simulink model "Hexapod_PD"  (R2026a)
settings: Solver=daessc  StopTime=ref.t(end)  FixedStep=2e-5
InitFcn:
  | startup
model workspace: external: MATLAB File Hexapod_DataFile.m (data not in the file)
undefined symbols (not defined in the file or in its folder): ref, robot, smiData, vc, X, Y, Z
libraries: sm_lib x805, nesl_utility x43
(part 7 of 15)

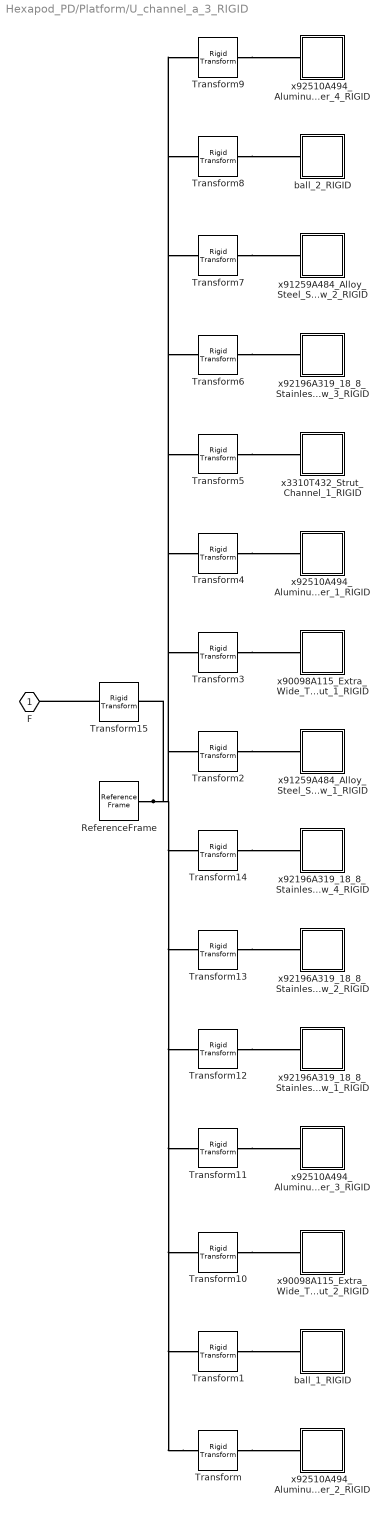
== system Hexapod_PD/Platform/U_channel_a_3_RIGID ==
  ReferenceFrame : sm_lib/Frames and Transforms/Reference Frame
  Transform : sm_lib/Frames and Transforms/Rigid Transform  RotationMethod=ArbitraryAxis  FollAlignAxisA=+X  BaseAlignAxisA=+Y  FollAlignAxisB=+Y  BaseAlignAxisB=+Z  RotationStandardAxis=+Z  RotationAngle=smiData.RigidTransform(213).angle  RotationAngleUnits=rad  RotationArbitraryAxis=smiData.RigidTransform(213).axis  RotationSequenceAxes=FollowerAxes  RotationSequence=XYX  RotationSequenceAngles=[0 0 0]  RotationSequenceAnglesUnits=deg  RotationMatrix=[1 0 0;0 1 0;0 0 1]  Quaternion=[1 0 0 0]  TranslationMethod=Cartesian  TranslationCartesianOffset=smiData.RigidTransform(213).translation  TranslationCartesianOffsetUnits=mm  TranslationStandardAxis=+Z  TranslationStandardOffset=0  TranslationStandardOffsetUnits=m  TranslationROffset=0  TranslationROffsetUnits=m  TranslationThetaOffset=0  TranslationThetaOffsetUnits=deg  TranslationZOffset=0  TranslationZOffsetUnits=m
  Transform1 : sm_lib/Frames and Transforms/Rigid Transform  RotationMethod=ArbitraryAxis  FollAlignAxisA=+X  BaseAlignAxisA=+Y  FollAlignAxisB=+Y  BaseAlignAxisB=+Z  RotationStandardAxis=+Z  RotationAngle=smiData.RigidTransform(214).angle  RotationAngleUnits=rad  RotationArbitraryAxis=smiData.RigidTransform(214).axis  RotationSequenceAxes=FollowerAxes  RotationSequence=XYX  RotationSequenceAngles=[0 0 0]  RotationSequenceAnglesUnits=deg  RotationMatrix=[1 0 0;0 1 0;0 0 1]  Quaternion=[1 0 0 0]  TranslationMethod=Cartesian  TranslationCartesianOffset=smiData.RigidTransform(214).translation  TranslationCartesianOffsetUnits=mm  TranslationStandardAxis=+Z  TranslationStandardOffset=0  TranslationStandardOffsetUnits=m  TranslationROffset=0  TranslationROffsetUnits=m  TranslationThetaOffset=0  TranslationThetaOffsetUnits=deg  TranslationZOffset=0  TranslationZOffsetUnits=m
  Transform10 : sm_lib/Frames and Transforms/Rigid Transform  RotationMethod=ArbitraryAxis  FollAlignAxisA=+X  BaseAlignAxisA=+Y  FollAlignAxisB=+Y  BaseAlignAxisB=+Z  RotationStandardAxis=+Z  RotationAngle=smiData.RigidTransform(223).angle  RotationAngleUnits=rad  RotationArbitraryAxis=smiData.RigidTransform(223).axis  RotationSequenceAxes=FollowerAxes  RotationSequence=XYX  RotationSequenceAngles=[0 0 0]  RotationSequenceAnglesUnits=deg  RotationMatrix=[1 0 0;0 1 0;0 0 1]  Quaternion=[1 0 0 0]  TranslationMethod=Cartesian  TranslationCartesianOffset=smiData.RigidTransform(223).translation  TranslationCartesianOffsetUnits=mm  TranslationStandardAxis=+Z  TranslationStandardOffset=0  TranslationStandardOffsetUnits=m  TranslationROffset=0  TranslationROffsetUnits=m  TranslationThetaOffset=0  TranslationThetaOffsetUnits=deg  TranslationZOffset=0  TranslationZOffsetUnits=m
  Transform11 : sm_lib/Frames and Transforms/Rigid Transform  RotationMethod=ArbitraryAxis  FollAlignAxisA=+X  BaseAlignAxisA=+Y  FollAlignAxisB=+Y  BaseAlignAxisB=+Z  RotationStandardAxis=+Z  RotationAngle=smiData.RigidTransform(224).angle  RotationAngleUnits=rad  RotationArbitraryAxis=smiData.RigidTransform(224).axis  RotationSequenceAxes=FollowerAxes  RotationSequence=XYX  RotationSequenceAngles=[0 0 0]  RotationSequenceAnglesUnits=deg  RotationMatrix=[1 0 0;0 1 0;0 0 1]  Quaternion=[1 0 0 0]  TranslationMethod=Cartesian  TranslationCartesianOffset=smiData.RigidTransform(224).translation  TranslationCartesianOffsetUnits=mm  TranslationStandardAxis=+Z  TranslationStandardOffset=0  TranslationStandardOffsetUnits=m  TranslationROffset=0  TranslationROffsetUnits=m  TranslationThetaOffset=0  TranslationThetaOffsetUnits=deg  TranslationZOffset=0  TranslationZOffsetUnits=m
  Transform12 : sm_lib/Frames and Transforms/Rigid Transform  RotationMethod=ArbitraryAxis  FollAlignAxisA=+X  BaseAlignAxisA=+Y  FollAlignAxisB=+Y  BaseAlignAxisB=+Z  RotationStandardAxis=+Z  RotationAngle=smiData.RigidTransform(225).angle  RotationAngleUnits=rad  RotationArbitraryAxis=smiData.RigidTransform(225).axis  RotationSequenceAxes=FollowerAxes  RotationSequence=XYX  RotationSequenceAngles=[0 0 0]  RotationSequenceAnglesUnits=deg  RotationMatrix=[1 0 0;0 1 0;0 0 1]  Quaternion=[1 0 0 0]  TranslationMethod=Cartesian  TranslationCartesianOffset=smiData.RigidTransform(225).translation  TranslationCartesianOffsetUnits=mm  TranslationStandardAxis=+Z  TranslationStandardOffset=0  TranslationStandardOffsetUnits=m  TranslationROffset=0  TranslationROffsetUnits=m  TranslationThetaOffset=0  TranslationThetaOffsetUnits=deg  TranslationZOffset=0  TranslationZOffsetUnits=m
  Transform13 : sm_lib/Frames and Transforms/Rigid Transform  RotationMethod=ArbitraryAxis  FollAlignAxisA=+X  BaseAlignAxisA=+Y  FollAlignAxisB=+Y  BaseAlignAxisB=+Z  RotationStandardAxis=+Z  RotationAngle=smiData.RigidTransform(226).angle  RotationAngleUnits=rad  RotationArbitraryAxis=smiData.RigidTransform(226).axis  RotationSequenceAxes=FollowerAxes  RotationSequence=XYX  RotationSequenceAngles=[0 0 0]  RotationSequenceAnglesUnits=deg  RotationMatrix=[1 0 0;0 1 0;0 0 1]  Quaternion=[1 0 0 0]  TranslationMethod=Cartesian  TranslationCartesianOffset=smiData.RigidTransform(226).translation  TranslationCartesianOffsetUnits=mm  TranslationStandardAxis=+Z  TranslationStandardOffset=0  TranslationStandardOffsetUnits=m  TranslationROffset=0  TranslationROffsetUnits=m  TranslationThetaOffset=0  TranslationThetaOffsetUnits=deg  TranslationZOffset=0  TranslationZOffsetUnits=m
  Transform14 : sm_lib/Frames and Transforms/Rigid Transform  RotationMethod=ArbitraryAxis  FollAlignAxisA=+X  BaseAlignAxisA=+Y  FollAlignAxisB=+Y  BaseAlignAxisB=+Z  RotationStandardAxis=+Z  RotationAngle=smiData.RigidTransform(227).angle  RotationAngleUnits=rad  RotationArbitraryAxis=smiData.RigidTransform(227).axis  RotationSequenceAxes=FollowerAxes  RotationSequence=XYX  RotationSequenceAngles=[0 0 0]  RotationSequenceAnglesUnits=deg  RotationMatrix=[1 0 0;0 1 0;0 0 1]  Quaternion=[1 0 0 0]  TranslationMethod=Cartesian  TranslationCartesianOffset=smiData.RigidTransform(227).translation  TranslationCartesianOffsetUnits=mm  TranslationStandardAxis=+Z  TranslationStandardOffset=0  TranslationStandardOffsetUnits=m  TranslationROffset=0  TranslationROffsetUnits=m  TranslationThetaOffset=0  TranslationThetaOffsetUnits=deg  TranslationZOffset=0  TranslationZOffsetUnits=m
  Transform15 : sm_lib/Frames and Transforms/Rigid Transform  RotationMethod=ArbitraryAxis  FollAlignAxisA=+X  BaseAlignAxisA=+Y  FollAlignAxisB=+Y  BaseAlignAxisB=+Z  RotationStandardAxis=+Z  RotationAngle=smiData.RigidTransform(228).angle  RotationAngleUnits=rad  RotationArbitraryAxis=smiData.RigidTransform(228).axis  RotationSequenceAxes=FollowerAxes  RotationSequence=XYX  RotationSequenceAngles=[0 0 0]  RotationSequenceAnglesUnits=deg  RotationMatrix=[1 0 0;0 1 0;0 0 1]  Quaternion=[1 0 0 0]  TranslationMethod=Cartesian  TranslationCartesianOffset=smiData.RigidTransform(228).translation  TranslationCartesianOffsetUnits=mm  TranslationStandardAxis=+Z  TranslationStandardOffset=0  TranslationStandardOffsetUnits=m  TranslationROffset=0  TranslationROffsetUnits=m  TranslationThetaOffset=0  TranslationThetaOffsetUnits=deg  TranslationZOffset=0  TranslationZOffsetUnits=m
  Transform2 : sm_lib/Frames and Transforms/Rigid Transform  RotationMethod=ArbitraryAxis  FollAlignAxisA=+X  BaseAlignAxisA=+Y  FollAlignAxisB=+Y  BaseAlignAxisB=+Z  RotationStandardAxis=+Z  RotationAngle=smiData.RigidTransform(215).angle  RotationAngleUnits=rad  RotationArbitraryAxis=smiData.RigidTransform(215).axis  RotationSequenceAxes=FollowerAxes  RotationSequence=XYX  RotationSequenceAngles=[0 0 0]  RotationSequenceAnglesUnits=deg  RotationMatrix=[1 0 0;0 1 0;0 0 1]  Quaternion=[1 0 0 0]  TranslationMethod=Cartesian  TranslationCartesianOffset=smiData.RigidTransform(215).translation  TranslationCartesianOffsetUnits=mm  TranslationStandardAxis=+Z  TranslationStandardOffset=0  TranslationStandardOffsetUnits=m  TranslationROffset=0  TranslationROffsetUnits=m  TranslationThetaOffset=0  TranslationThetaOffsetUnits=deg  TranslationZOffset=0  TranslationZOffsetUnits=m
  Transform3 : sm_lib/Frames and Transforms/Rigid Transform  RotationMethod=ArbitraryAxis  FollAlignAxisA=+X  BaseAlignAxisA=+Y  FollAlignAxisB=+Y  BaseAlignAxisB=+Z  RotationStandardAxis=+Z  RotationAngle=smiData.RigidTransform(216).angle  RotationAngleUnits=rad  RotationArbitraryAxis=smiData.RigidTransform(216).axis  RotationSequenceAxes=FollowerAxes  RotationSequence=XYX  RotationSequenceAngles=[0 0 0]  RotationSequenceAnglesUnits=deg  RotationMatrix=[1 0 0;0 1 0;0 0 1]  Quaternion=[1 0 0 0]  TranslationMethod=Cartesian  TranslationCartesianOffset=smiData.RigidTransform(216).translation  TranslationCartesianOffsetUnits=mm  TranslationStandardAxis=+Z  TranslationStandardOffset=0  TranslationStandardOffsetUnits=m  TranslationROffset=0  TranslationROffsetUnits=m  TranslationThetaOffset=0  TranslationThetaOffsetUnits=deg  TranslationZOffset=0  TranslationZOffsetUnits=m
  Transform4 : sm_lib/Frames and Transforms/Rigid Transform  RotationMethod=ArbitraryAxis  FollAlignAxisA=+X  BaseAlignAxisA=+Y  FollAlignAxisB=+Y  BaseAlignAxisB=+Z  RotationStandardAxis=+Z  RotationAngle=smiData.RigidTransform(217).angle  RotationAngleUnits=rad  RotationArbitraryAxis=smiData.RigidTransform(217).axis  RotationSequenceAxes=FollowerAxes  RotationSequence=XYX  RotationSequenceAngles=[0 0 0]  RotationSequenceAnglesUnits=deg  RotationMatrix=[1 0 0;0 1 0;0 0 1]  Quaternion=[1 0 0 0]  TranslationMethod=Cartesian  TranslationCartesianOffset=smiData.RigidTransform(217).translation  TranslationCartesianOffsetUnits=mm  TranslationStandardAxis=+Z  TranslationStandardOffset=0  TranslationStandardOffsetUnits=m  TranslationROffset=0  TranslationROffsetUnits=m  TranslationThetaOffset=0  TranslationThetaOffsetUnits=deg  TranslationZOffset=0  TranslationZOffsetUnits=m
  Transform5 : sm_lib/Frames and Transforms/Rigid Transform  RotationMethod=ArbitraryAxis  FollAlignAxisA=+X  BaseAlignAxisA=+Y  FollAlignAxisB=+Y  BaseAlignAxisB=+Z  RotationStandardAxis=+Z  RotationAngle=smiData.RigidTransform(218).angle  RotationAngleUnits=rad  RotationArbitraryAxis=smiData.RigidTransform(218).axis  RotationSequenceAxes=FollowerAxes  RotationSequence=XYX  RotationSequenceAngles=[0 0 0]  RotationSequenceAnglesUnits=deg  RotationMatrix=[1 0 0;0 1 0;0 0 1]  Quaternion=[1 0 0 0]  TranslationMethod=Cartesian  TranslationCartesianOffset=smiData.RigidTransform(218).translation  TranslationCartesianOffsetUnits=mm  TranslationStandardAxis=+Z  TranslationStandardOffset=0  TranslationStandardOffsetUnits=m  TranslationROffset=0  TranslationROffsetUnits=m  TranslationThetaOffset=0  TranslationThetaOffsetUnits=deg  TranslationZOffset=0  TranslationZOffsetUnits=m
  Transform6 : sm_lib/Frames and Transforms/Rigid Transform  RotationMethod=ArbitraryAxis  FollAlignAxisA=+X  BaseAlignAxisA=+Y  FollAlignAxisB=+Y  BaseAlignAxisB=+Z  RotationStandardAxis=+Z  RotationAngle=smiData.RigidTransform(219).angle  RotationAngleUnits=rad  RotationArbitraryAxis=smiData.RigidTransform(219).axis  RotationSequenceAxes=FollowerAxes  RotationSequence=XYX  RotationSequenceAngles=[0 0 0]  RotationSequenceAnglesUnits=deg  RotationMatrix=[1 0 0;0 1 0;0 0 1]  Quaternion=[1 0 0 0]  TranslationMethod=Cartesian  TranslationCartesianOffset=smiData.RigidTransform(219).translation  TranslationCartesianOffsetUnits=mm  TranslationStandardAxis=+Z  TranslationStandardOffset=0  TranslationStandardOffsetUnits=m  TranslationROffset=0  TranslationROffsetUnits=m  TranslationThetaOffset=0  TranslationThetaOffsetUnits=deg  TranslationZOffset=0  TranslationZOffsetUnits=m
  Transform7 : sm_lib/Frames and Transforms/Rigid Transform  RotationMethod=ArbitraryAxis  FollAlignAxisA=+X  BaseAlignAxisA=+Y  FollAlignAxisB=+Y  BaseAlignAxisB=+Z  RotationStandardAxis=+Z  RotationAngle=smiData.RigidTransform(220).angle  RotationAngleUnits=rad  RotationArbitraryAxis=smiData.RigidTransform(220).axis  RotationSequenceAxes=FollowerAxes  RotationSequence=XYX  RotationSequenceAngles=[0 0 0]  RotationSequenceAnglesUnits=deg  RotationMatrix=[1 0 0;0 1 0;0 0 1]  Quaternion=[1 0 0 0]  TranslationMethod=Cartesian  TranslationCartesianOffset=smiData.RigidTransform(220).translation  TranslationCartesianOffsetUnits=mm  TranslationStandardAxis=+Z  TranslationStandardOffset=0  TranslationStandardOffsetUnits=m  TranslationROffset=0  TranslationROffsetUnits=m  TranslationThetaOffset=0  TranslationThetaOffsetUnits=deg  TranslationZOffset=0  TranslationZOffsetUnits=m
  Transform8 : sm_lib/Frames and Transforms/Rigid Transform  RotationMethod=ArbitraryAxis  FollAlignAxisA=+X  BaseAlignAxisA=+Y  FollAlignAxisB=+Y  BaseAlignAxisB=+Z  RotationStandardAxis=+Z  RotationAngle=smiData.RigidTransform(221).angle  RotationAngleUnits=rad  RotationArbitraryAxis=smiData.RigidTransform(221).axis  RotationSequenceAxes=FollowerAxes  RotationSequence=XYX  RotationSequenceAngles=[0 0 0]  RotationSequenceAnglesUnits=deg  RotationMatrix=[1 0 0;0 1 0;0 0 1]  Quaternion=[1 0 0 0]  TranslationMethod=Cartesian  TranslationCartesianOffset=smiData.RigidTransform(221).translation  TranslationCartesianOffsetUnits=mm  TranslationStandardAxis=+Z  TranslationStandardOffset=0  TranslationStandardOffsetUnits=m  TranslationROffset=0  TranslationROffsetUnits=m  TranslationThetaOffset=0  TranslationThetaOffsetUnits=deg  TranslationZOffset=0  TranslationZOffsetUnits=m
  Transform9 : sm_lib/Frames and Transforms/Rigid Transform  RotationMethod=ArbitraryAxis  FollAlignAxisA=+X  BaseAlignAxisA=+Y  FollAlignAxisB=+Y  BaseAlignAxisB=+Z  RotationStandardAxis=+Z  RotationAngle=smiData.RigidTransform(222).angle  RotationAngleUnits=rad  RotationArbitraryAxis=smiData.RigidTransform(222).axis  RotationSequenceAxes=FollowerAxes  RotationSequence=XYX  RotationSequenceAngles=[0 0 0]  RotationSequenceAnglesUnits=deg  RotationMatrix=[1 0 0;0 1 0;0 0 1]  Quaternion=[1 0 0 0]  TranslationMethod=Cartesian  TranslationCartesianOffset=smiData.RigidTransform(222).translation  TranslationCartesianOffsetUnits=mm  TranslationStandardAxis=+Z  TranslationStandardOffset=0  TranslationStandardOffsetUnits=m  TranslationROffset=0  TranslationROffsetUnits=m  TranslationThetaOffset=0  TranslationThetaOffsetUnits=deg  TranslationZOffset=0  TranslationZOffsetUnits=m
  ball_1_RIGID : Subsystem
  ball_2_RIGID : Subsystem
  x3310T432_Strut_Channel_1_RIGID : Subsystem
  x90098A115_Extra_Wide_Thin_Nylon_Insert_Locknut_1_RIGID : Subsystem
  x90098A115_Extra_Wide_Thin_Nylon_Insert_Locknut_2_RIGID : Subsystem
  x91259A484_Alloy_Steel_Shoulder_Screw_1_RIGID : Subsystem
  x91259A484_Alloy_Steel_Shoulder_Screw_2_RIGID : Subsystem
  x92196A319_18_8_Stainless_Steel_Socket_Head_Screw_1_RIGID : Subsystem
  x92196A319_18_8_Stainless_Steel_Socket_Head_Screw_2_RIGID : Subsystem
  x92196A319_18_8_Stainless_Steel_Socket_Head_Screw_3_RIGID : Subsystem
  x92196A319_18_8_Stainless_Steel_Socket_Head_Screw_4_RIGID : Subsystem
  x92510A494_Aluminum_Unthreaded_Spacer_1_RIGID : Subsystem
  x92510A494_Aluminum_Unthreaded_Spacer_2_RIGID : Subsystem
  x92510A494_Aluminum_Unthreaded_Spacer_3_RIGID : Subsystem
  x92510A494_Aluminum_Unthreaded_Spacer_4_RIGID : Subsystem
  F : PMIOPort  Side=Right
  connections:
  Transform/RConn1 -- x92510A494_Aluminum_Unthreaded_Spacer_2_RIGID/LConn1
  Transform1/RConn1 -- ball_1_RIGID/LConn1
  Transform10/RConn1 -- x90098A115_Extra_Wide_Thin_Nylon_Insert_Locknut_2_RIGID/LConn1
  Transform11/RConn1 -- x92510A494_Aluminum_Unthreaded_Spacer_3_RIGID/LConn1
  Transform12/RConn1 -- x92196A319_18_8_Stainless_Steel_Socket_Head_Screw_1_RIGID/LConn1
  Transform13/RConn1 -- x92196A319_18_8_Stainless_Steel_Socket_Head_Screw_2_RIGID/LConn1
  Transform14/RConn1 -- x92196A319_18_8_Stainless_Steel_Socket_Head_Screw_4_RIGID/LConn1
  Transform/LConn1 -- ReferenceFrame/RConn1 -- Transform1/LConn1 -- Transform10/LConn1 -- Transform11/LConn1 -- Transform12/LConn1 -- Transform13/LConn1 -- Transform14/LConn1 -- Transform15/RConn1 -- Transform2/LConn1 -- Transform3/LConn1 -- Transform4/LConn1 -- Transform5/LConn1 -- Transform6/LConn1 -- Transform7/LConn1 -- Transform8/LConn1 -- Transform9/LConn1
  Transform15/LConn1 -- F/RConn1
  Transform2/RConn1 -- x91259A484_Alloy_Steel_Shoulder_Screw_1_RIGID/LConn1
  Transform3/RConn1 -- x90098A115_Extra_Wide_Thin_Nylon_Insert_Locknut_1_RIGID/LConn1
  Transform4/RConn1 -- x92510A494_Aluminum_Unthreaded_Spacer_1_RIGID/LConn1
  Transform5/RConn1 -- x3310T432_Strut_Channel_1_RIGID/LConn1
  Transform6/RConn1 -- x92196A319_18_8_Stainless_Steel_Socket_Head_Screw_3_RIGID/LConn1
  Transform7/RConn1 -- x91259A484_Alloy_Steel_Shoulder_Screw_2_RIGID/LConn1
  Transform8/RConn1 -- ball_2_RIGID/LConn1
  Transform9/RConn1 -- x92510A494_Aluminum_Unthreaded_Spacer_4_RIGID/LConn1

== system Hexapod_PD/Platform pose logger/g ==
  Ina : Inport
  Demux : Demux  Outputs=3
  Mux1 : Mux  Inputs=3
  g : Bias  Bias=robot.g  SaturateOnIntegerOverflow=off
  Outa : Outport
  wires:
  Demux/1 -> Mux1/1
  Demux/3 -> g/1
  Mux1/1 -> Outa/1
  g/1 -> Mux1/3
  Demux/2 -> Mux1/2
  Ina/1 -> Demux/1

== system Hexapod_PD/Revolute Joints/PD controller1 ==
  clock : Inport
  Add : Sum
  Constant : Constant  Value=deg2rad(smiData.RevoluteJoint(1).Rz.Pos)
  D gain : Gain  Gain=vc.Kd
  Differentiator : TransferFcn  Numerator=[vc.wf 0]  Denominator=[1 vc.wf]
  FF gin : Gain  Gain=vc.Kv
  Gain : Gain  Gain=-1
  Integrator : Integrator
  P gain : Gain  Gain=vc.Kp
  Sum : Sum  Inputs=|++-
  Sum1 : Sum  Inputs=|+-
  Velocity Plant : TransferFcn  Numerator=[robot.drive.a]  Denominator=[1 robot.drive.b]
  du : Lookup_n-D  NumberOfTableDimensions=1  BreakpointsForDimension1=ref.t  Table=ref.qd(:,1)  InterpMethod=Cubic spline  InternalRulePriority=Speed  RndMeth=Simplest
  u : Lookup_n-D  NumberOfTableDimensions=1  BreakpointsForDimension1=ref.t  Table=ref.q(:,1)  InterpMethod=Cubic spline  InternalRulePriority=Speed  RndMeth=Simplest
  y : Outport
  wires:
  P gain/1 -> Sum/2
  Sum/1 -> Velocity Plant/1
  Sum1/1 -> P gain/1
  Velocity Plant/1 -> Integrator/1
  D gain/1 -> Sum/3
  Differentiator/1 -> D gain/1
  du/1 -> FF gin/1  "omega ref"
  FF gin/1 -> Sum/1
  clock/1 -> u/1, du/1
  u/1 -> Sum1/1  "theta ref"
  Integrator/1 -> Gain/1, Sum1/2, Differentiator/1
  Add/1 -> y/1
  Gain/1 -> Add/2
  Constant/1 -> Add/1

== system Hexapod_PD/Revolute Joints/PD controller2 ==
  clock : Inport
  Add : Sum
  Constant : Constant  Value=deg2rad(smiData.RevoluteJoint(2).Rz.Pos)
  D gain : Gain  Gain=vc.Kd
  Differentiator : TransferFcn  Numerator=[vc.wf 0]  Denominator=[1 vc.wf]
  FF gin : Gain  Gain=vc.Kv
  Gain : Gain
  Integrator : Integrator
  P gain : Gain  Gain=vc.Kp
  Sum : Sum  Inputs=|++-
  Sum1 : Sum  Inputs=|+-
  Velocity Plant : TransferFcn  Numerator=[robot.drive.a]  Denominator=[1 robot.drive.b]
  du : Lookup_n-D  NumberOfTableDimensions=1  BreakpointsForDimension1=ref.t  Table=ref.qd(:,2)  InterpMethod=Cubic spline  InternalRulePriority=Speed  RndMeth=Simplest
  u : Lookup_n-D  NumberOfTableDimensions=1  BreakpointsForDimension1=ref.t  Table=ref.q(:,2)  InterpMethod=Cubic spline  InternalRulePriority=Speed  RndMeth=Simplest
  y : Outport
  wires:
  P gain/1 -> Sum/2
  Sum/1 -> Velocity Plant/1
  Sum1/1 -> P gain/1
  Velocity Plant/1 -> Integrator/1
  D gain/1 -> Sum/3
  Differentiator/1 -> D gain/1
  du/1 -> FF gin/1  "v ref"
  FF gin/1 -> Sum/1
  clock/1 -> u/1, du/1
  u/1 -> Sum1/1
  Integrator/1 -> Gain/1, Sum1/2, Differentiator/1
  Gain/1 -> Add/1
  Constant/1 -> Add/2
  Add/1 -> y/1

== system Hexapod_PD/Revolute Joints/PD controller3 ==
  clock : Inport
  Add : Sum
  Constant : Constant  Value=deg2rad(smiData.RevoluteJoint(5).Rz.Pos)
  D gain : Gain  Gain=vc.Kd
  Differentiator : TransferFcn  Numerator=[vc.wf 0]  Denominator=[1 vc.wf]
  FF gin : Gain  Gain=vc.Kv
  Gain : Gain  Gain=-1
  Integrator : Integrator
  P gain : Gain  Gain=vc.Kp
  Sum : Sum  Inputs=|++-
  Sum1 : Sum  Inputs=|+-
  Velocity Plant : TransferFcn  Numerator=[robot.drive.a]  Denominator=[1 robot.drive.b]
  du : Lookup_n-D  NumberOfTableDimensions=1  BreakpointsForDimension1=ref.t  Table=ref.qd(:,3)  InterpMethod=Cubic spline  InternalRulePriority=Speed  RndMeth=Simplest
  u : Lookup_n-D  NumberOfTableDimensions=1  BreakpointsForDimension1=ref.t  Table=ref.q(:,3)  InterpMethod=Cubic spline  InternalRulePriority=Speed  RndMeth=Simplest
  y : Outport
  wires:
  P gain/1 -> Sum/2
  Sum/1 -> Velocity Plant/1
  Sum1/1 -> P gain/1
  Velocity Plant/1 -> Integrator/1
  D gain/1 -> Sum/3
  Differentiator/1 -> D gain/1
  du/1 -> FF gin/1  "v ref"
  FF gin/1 -> Sum/1
  clock/1 -> u/1, du/1
  u/1 -> Sum1/1
  Integrator/1 -> Gain/1, Sum1/2, Differentiator/1
  Gain/1 -> Add/1
  Constant/1 -> Add/2
  Add/1 -> y/1

== system Hexapod_PD/Revolute Joints/PD controller4 ==
  clock : Inport
  Add : Sum
  Constant : Constant  Value=deg2rad(smiData.RevoluteJoint(6).Rz.Pos)
  D gain : Gain  Gain=vc.Kd
  Differentiator : TransferFcn  Numerator=[vc.wf 0]  Denominator=[1 vc.wf]
  FF gin : Gain  Gain=vc.Kv
  Gain : Gain
  Integrator : Integrator
  P gain : Gain  Gain=vc.Kp
  Sum : Sum  Inputs=|++-
  Sum1 : Sum  Inputs=|+-
  Velocity Plant : TransferFcn  Numerator=[robot.drive.a]  Denominator=[1 robot.drive.b]
  du : Lookup_n-D  NumberOfTableDimensions=1  BreakpointsForDimension1=ref.t  Table=ref.qd(:,4)  InterpMethod=Cubic spline  InternalRulePriority=Speed  RndMeth=Simplest
  u : Lookup_n-D  NumberOfTableDimensions=1  BreakpointsForDimension1=ref.t  Table=ref.q(:,4)  InterpMethod=Cubic spline  InternalRulePriority=Speed  RndMeth=Simplest
  y : Outport
  wires:
  P gain/1 -> Sum/2
  Sum/1 -> Velocity Plant/1
  Sum1/1 -> P gain/1
  Velocity Plant/1 -> Integrator/1
  D gain/1 -> Sum/3
  Differentiator/1 -> D gain/1
  du/1 -> FF gin/1  "v ref"
  FF gin/1 -> Sum/1
  clock/1 -> u/1, du/1
  u/1 -> Sum1/1
  Integrator/1 -> Gain/1, Sum1/2, Differentiator/1
  Gain/1 -> Add/1
  Constant/1 -> Add/2
  Add/1 -> y/1

== system Hexapod_PD/Revolute Joints/PD controller5 ==
  clock : Inport
  Add : Sum
  Constant : Constant  Value=deg2rad(smiData.RevoluteJoint(3).Rz.Pos)
  D gain : Gain  Gain=vc.Kd
  Differentiator : TransferFcn  Numerator=[vc.wf 0]  Denominator=[1 vc.wf]
  FF gin : Gain  Gain=vc.Kv
  Gain : Gain  Gain=-1
  Integrator : Integrator
  P gain : Gain  Gain=vc.Kp
  Sum : Sum  Inputs=|++-
  Sum1 : Sum  Inputs=|+-
  Velocity Plant : TransferFcn  Numerator=[robot.drive.a]  Denominator=[1 robot.drive.b]
  du : Lookup_n-D  NumberOfTableDimensions=1  BreakpointsForDimension1=ref.t  Table=ref.qd(:,5)  InterpMethod=Cubic spline  InternalRulePriority=Speed  RndMeth=Simplest
  u : Lookup_n-D  NumberOfTableDimensions=1  BreakpointsForDimension1=ref.t  Table=ref.q(:,5)  InterpMethod=Cubic spline  InternalRulePriority=Speed  RndMeth=Simplest
  y : Outport
  wires:
  P gain/1 -> Sum/2
  Sum/1 -> Velocity Plant/1
  Sum1/1 -> P gain/1
  Velocity Plant/1 -> Integrator/1
  D gain/1 -> Sum/3
  Differentiator/1 -> D gain/1
  du/1 -> FF gin/1  "v ref"
  FF gin/1 -> Sum/1
  clock/1 -> u/1, du/1
  u/1 -> Sum1/1
  Integrator/1 -> Gain/1, Sum1/2, Differentiator/1
  Gain/1 -> Add/1
  Constant/1 -> Add/2
  Add/1 -> y/1

== system Hexapod_PD/Revolute Joints/PD controller6 ==
  clock : Inport
  Add : Sum
  Constant : Constant  Value=deg2rad(smiData.RevoluteJoint(4).Rz.Pos)
  D gain : Gain  Gain=vc.Kd
  Differentiator : TransferFcn  Numerator=[vc.wf 0]  Denominator=[1 vc.wf]
  FF gin : Gain  Gain=vc.Kv
  Gain : Gain
  Integrator : Integrator
  P gain : Gain  Gain=vc.Kp
  Sum : Sum  Inputs=|++-
  Sum1 : Sum  Inputs=|+-
  Velocity Plant : TransferFcn  Numerator=[robot.drive.a]  Denominator=[1 robot.drive.b]
  du : Lookup_n-D  NumberOfTableDimensions=1  BreakpointsForDimension1=ref.t  Table=ref.qd(:,6)  InterpMethod=Cubic spline  InternalRulePriority=Speed  RndMeth=Simplest
  u : Lookup_n-D  NumberOfTableDimensions=1  BreakpointsForDimension1=ref.t  Table=ref.q(:,6)  InterpMethod=Cubic spline  InternalRulePriority=Speed  RndMeth=Simplest
  y : Outport
  wires:
  P gain/1 -> Sum/2
  Sum/1 -> Velocity Plant/1
  Sum1/1 -> P gain/1
  Velocity Plant/1 -> Integrator/1
  D gain/1 -> Sum/3
  Differentiator/1 -> D gain/1
  du/1 -> FF gin/1  "v ref"
  FF gin/1 -> Sum/1
  clock/1 -> u/1, du/1
  u/1 -> Sum1/1
  Integrator/1 -> Gain/1, Sum1/2, Differentiator/1
  Gain/1 -> Add/1
  Constant/1 -> Add/2
  Add/1 -> y/1

== system Hexapod_PD/Revolute Joints/Subsystem ==
  Gain2 : Gain  Gain=-1
  MotorFrametoBodyFrame3 : Subsystem
  Mux2 : Mux
  PS-Simulink Converter{8..11} (4 alike) : nesl_utility/PS-Simulink Converter  PhysicalDomain=network_engine_domain  SubClassName=ps_output  LeftPortType=input  RightPortType=output  PseudoPeriodic=off  Frequencies=[]  VectorFormat=inherit  Unit=inherit  AffineConversion=off
  q : PMIOPort  Side=Left
  w : PMIOPort  Port=2  Side=Left
  b : PMIOPort  Port=3  Side=Left
  t : PMIOPort  Port=4  Side=Left
  3 : Outport
  wires:
  PS-Simulink Converter8/1 -> MotorFrametoBodyFrame3/1(M)
  PS-Simulink Converter9/1 -> Mux2/2
  PS-Simulink Converter10/1 -> Mux2/3
  MotorFrametoBodyFrame3/1(B) -> Mux2/1
  Mux2/1 -> Gain2/1
  PS-Simulink Converter11/1 -> Mux2/4
  Gain2/1 -> 3/1
  connections:
  t/RConn1 -- PS-Simulink Converter11/LConn1
  b/RConn1 -- PS-Simulink Converter10/LConn1
  q/RConn1 -- PS-Simulink Converter8/LConn1
  w/RConn1 -- PS-Simulink Converter9/LConn1

== system Hexapod_PD/Revolute Joints/Subsystem10 ==
  Gain3 : Gain  Gain=-1
  MotorFrametoBodyFrame5 : Subsystem
  Mux4 : Mux
  PS-Simulink Converter{16..19} (4 alike) : nesl_utility/PS-Simulink Converter  PhysicalDomain=network_engine_domain  SubClassName=ps_output  LeftPortType=input  RightPortType=output  PseudoPeriodic=off  Frequencies=[]  VectorFormat=inherit  Unit=inherit  AffineConversion=off
  q : PMIOPort  Side=Left
  w : PMIOPort  Port=2  Side=Left
  b : PMIOPort  Port=3  Side=Left
  t : PMIOPort  Port=4  Side=Left
  5 : Outport
  wires:
  PS-Simulink Converter17/1 -> Mux4/4
  PS-Simulink Converter16/1 -> Mux4/3
  Mux4/1 -> Gain3/1
  PS-Simulink Converter18/1 -> MotorFrametoBodyFrame5/1(M)
  PS-Simulink Converter19/1 -> Mux4/2
  MotorFrametoBodyFrame5/1(B) -> Mux4/1
  Gain3/1 -> 5/1
  connections:
  w/RConn1 -- PS-Simulink Converter19/LConn1
  t/RConn1 -- PS-Simulink Converter17/LConn1
  b/RConn1 -- PS-Simulink Converter16/LConn1
  q/RConn1 -- PS-Simulink Converter18/LConn1

== system Hexapod_PD/Revolute Joints/Subsystem11 ==
  MotorFrametoBodyFrame6 : Subsystem
  Mux5 : Mux
  PS-Simulink Converter{20..23} (4 alike) : nesl_utility/PS-Simulink Converter  PhysicalDomain=network_engine_domain  SubClassName=ps_output  LeftPortType=input  RightPortType=output  PseudoPeriodic=off  Frequencies=[]  VectorFormat=inherit  Unit=inherit  AffineConversion=off
  q : PMIOPort  Side=Left
  w : PMIOPort  Port=2  Side=Left
  b : PMIOPort  Port=3  Side=Left
  t : PMIOPort  Port=4  Side=Left
  6 : Outport
  wires:
  PS-Simulink Converter20/1 -> Mux5/3
  PS-Simulink Converter23/1 -> Mux5/2
  PS-Simulink Converter21/1 -> Mux5/4
  PS-Simulink Converter22/1 -> MotorFrametoBodyFrame6/1(M)
  MotorFrametoBodyFrame6/1(B) -> Mux5/1
  Mux5/1 -> 6/1
  connections:
  w/RConn1 -- PS-Simulink Converter23/LConn1
  t/RConn1 -- PS-Simulink Converter21/LConn1
  q/RConn1 -- PS-Simulink Converter22/LConn1
  b/RConn1 -- PS-Simulink Converter20/LConn1

== system Hexapod_PD/Revolute Joints/Subsystem7 ==
  Gain1 : Gain  Gain=-1
  MotorFrametoBodyFrame1 : Subsystem
  Mux : Mux
  PS-Simulink Converter{,1..3} (4 alike) : nesl_utility/PS-Simulink Converter  PhysicalDomain=network_engine_domain  SubClassName=ps_output  LeftPortType=input  RightPortType=output  PseudoPeriodic=off  Frequencies=[]  VectorFormat=inherit  Unit=inherit  AffineConversion=off
  q : PMIOPort  Side=Left
  w : PMIOPort  Port=2  Side=Left
  b : PMIOPort  Port=3  Side=Left
  t : PMIOPort  Port=4  Side=Left
  1 : Outport
  wires:
  Mux/1 -> Gain1/1
  PS-Simulink Converter/1 -> MotorFrametoBodyFrame1/1(M)
  PS-Simulink Converter3/1 -> Mux/4
  MotorFrametoBodyFrame1/1(B) -> Mux/1
  PS-Simulink Converter2/1 -> Mux/3
  Gain1/1 -> 1/1
  PS-Simulink Converter1/1 -> Mux/2
  connections:
  w/RConn1 -- PS-Simulink Converter1/LConn1
  q/RConn1 -- PS-Simulink Converter/LConn1
  t/RConn1 -- PS-Simulink Converter3/LConn1
  b/RConn1 -- PS-Simulink Converter2/LConn1

== system Hexapod_PD/Revolute Joints/Subsystem8 ==
  MotorFrametoBodyFrame2 : Subsystem
  Mux1 : Mux
  PS-Simulink Converter{4..7} (4 alike) : nesl_utility/PS-Simulink Converter  PhysicalDomain=network_engine_domain  SubClassName=ps_output  LeftPortType=input  RightPortType=output  PseudoPeriodic=off  Frequencies=[]  VectorFormat=inherit  Unit=inherit  AffineConversion=off
  q : PMIOPort  Side=Left
  w : PMIOPort  Port=2  Side=Left
  b : PMIOPort  Port=3  Side=Left
  t : PMIOPort  Port=4  Side=Left
  2 : Outport
  wires:
  MotorFrametoBodyFrame2/1(B) -> Mux1/1
  PS-Simulink Converter4/1 -> MotorFrametoBodyFrame2/1(M)
  PS-Simulink Converter6/1 -> Mux1/3
  PS-Simulink Converter5/1 -> Mux1/2
  PS-Simulink Converter7/1 -> Mux1/4
  Mux1/1 -> 2/1
  connections:
  q/RConn1 -- PS-Simulink Converter4/LConn1
  w/RConn1 -- PS-Simulink Converter5/LConn1
  b/RConn1 -- PS-Simulink Converter6/LConn1
  t/RConn1 -- PS-Simulink Converter7/LConn1

== system Hexapod_PD/Revolute Joints/Subsystem9 ==
  MotorFrametoBodyFrame4 : Subsystem
  Mux3 : Mux
  PS-Simulink Converter{12..15} (4 alike) : nesl_utility/PS-Simulink Converter  PhysicalDomain=network_engine_domain  SubClassName=ps_output  LeftPortType=input  RightPortType=output  PseudoPeriodic=off  Frequencies=[]  VectorFormat=inherit  Unit=inherit  AffineConversion=off
  q : PMIOPort  Side=Left
  w : PMIOPort  Port=2  Side=Left
  b : PMIOPort  Port=3  Side=Left
  t : PMIOPort  Port=4  Side=Left
  4 : Outport
  wires:
  PS-Simulink Converter12/1 -> Mux3/3
  PS-Simulink Converter15/1 -> Mux3/2
  PS-Simulink Converter13/1 -> Mux3/4
  PS-Simulink Converter14/1 -> MotorFrametoBodyFrame4/1(M)
  MotorFrametoBodyFrame4/1(B) -> Mux3/1
  Mux3/1 -> 4/1
  connections:
  w/RConn1 -- PS-Simulink Converter15/LConn1
  t/RConn1 -- PS-Simulink Converter13/LConn1
  q/RConn1 -- PS-Simulink Converter14/LConn1
  b/RConn1 -- PS-Simulink Converter12/LConn1

== system Hexapod_PD/Spherical Joints/HeimJoint_No_Ball_1_RIGID1 ==
  ReferenceFrame : sm_lib/Frames and Transforms/Reference Frame
  Solid : sm_lib/Body Elements/File Solid  ExtGeomFileName=6960T431_Super-Swivel Ball Joint Rod End No Ball_6960T431_sldprt.STEP  UnitType=FromFile  ExtGeomFileUnits=m  StepReaderType=HEX  ExportConvexHullGeometry=off  InertiaType=Custom  BasedOnType=DensityFromFile  Density=1000  DensityUnits=kg/m^3  Mass=smiData.Solid(20).mass  MassUnits=kg  CenterOfMass=smiData.Solid(20).CoM  CenterOfMassUnits=in  MomentsOfInertia=smiData.Solid(20).MoI  MomentsOfInertiaUnits=kg*in^2  ProductsOfInertia=smiData.Solid(20).PoI  ProductsOfInertiaUnits=kg*in^2  GraphicType=FromGeometry  MarkerShape=Sphere  MarkerSize=10  GraphicVisPropType=SimpleVisualProperties  GraphicDiffuseColor=smiData.Solid(20).color  GraphicOpacity=smiData.Solid(20).opacity  GraphicSpecularColor=[0.5 0.5 0.5 1.0]  GraphicAmbientColor=[0.15 0.15 0.15 1.0]  GraphicEmissiveColor=[0.0 0.0 0.0 1.0]  GraphicShininess=75  DoExposeReferenceFrame=on  SerializedFrames=|
      | <Frames>
      | 
      |   <Frame>
      |     <Id>Frame1</Id>
      |     <Value>
      |       <Name>B</Name>
      |       <Origin>
      |         <Source>GeometricFeature</Source>
      |         <FeatureName>circular curve 99</FeatureName>
      |       </Origin>
      |       <PrimaryAxis>
      |         <DefinedDirection>+Z</DefinedDirection>
      |         <Source>ReferenceFrame</Source>
      |         <SourceDirection>+Z</SourceDirection>
      |         <FeatureName></FeatureName>
      |       </PrimaryAxis>
      |       <SecondaryAxis>
      |         <DefinedDirection>-X</DefinedDirection>
      |         <Source>GeometricFeature</Source>
      |         <SourceDirection>+X</SourceDirection>
      |         <FeatureName>segment 73</FeatureName>
      |       </SecondaryAxis>
      |     </Value>
      |   </Frame>
      | 
      | </Frames>
  Solid1 : sm_lib/Body Elements/File Solid  ExtGeomFileName=6960T432_Super-Swivel Ball Joint Rod End No Ball_6960T432_sldprt.STEP  UnitType=FromFile  ExtGeomFileUnits=m  StepReaderType=HEX  ExportConvexHullGeometry=off  InertiaType=Custom  BasedOnType=DensityFromFile  Density=1000  DensityUnits=kg/m^3  Mass=smiData.Solid(21).mass  MassUnits=kg  CenterOfMass=smiData.Solid(21).CoM  CenterOfMassUnits=in  MomentsOfInertia=smiData.Solid(21).MoI  MomentsOfInertiaUnits=kg*in^2  ProductsOfInertia=smiData.Solid(21).PoI  ProductsOfInertiaUnits=kg*in^2  GraphicType=FromGeometry  MarkerShape=Sphere  MarkerSize=10  GraphicVisPropType=SimpleVisualProperties  GraphicDiffuseColor=smiData.Solid(21).color  GraphicOpacity=smiData.Solid(21).opacity  GraphicSpecularColor=[0.5 0.5 0.5 1.0]  GraphicAmbientColor=[0.15 0.15 0.15 1.0]  GraphicEmissiveColor=[0.0 0.0 0.0 1.0]  GraphicShininess=75  DoExposeReferenceFrame=on  SerializedFrames=|
      | <Frames>
      | 
      |   <Frame>
      |     <Id>Frame1</Id>
      |     <Value>
      |       <Name>T</Name>
      |       <Origin>
      |         <Source>GeometricFeature</Source>
      |         <FeatureName>spherical surface 2</FeatureName>
      |       </Origin>
      |       <PrimaryAxis>
      |         <DefinedDirection>+Z</DefinedDirection>
      |         <Source>ReferenceFrame</Source>
      |         <SourceDirection>+Z</SourceDirection>
      |         <FeatureName></FeatureName>
      |       </PrimaryAxis>
      |       <SecondaryAxis>
      |         <DefinedDirection>+X</DefinedDirection>
      |         <Source>GeometricFeature</Source>
      |         <SourceDirection>+X</SourceDirection>
      |         <FeatureName>segment 75</FeatureName>
      |       </SecondaryAxis>
      |     </Value>
      |   </Frame>
      | 
      | </Frames>
  Solid2 : sm_lib/Body Elements/File Solid  ExtGeomFileName=8422N111_18-8 Stainless Steel Turnbuckle-Style Connecting Rod_8422N111_sldprt.STEP  UnitType=FromFile  ExtGeomFileUnits=m  StepReaderType=HEX  ExportConvexHullGeometry=off  InertiaType=Custom  BasedOnType=DensityFromFile  Density=1000  DensityUnits=kg/m^3  Mass=smiData.Solid(19).mass  MassUnits=kg  CenterOfMass=smiData.Solid(19).CoM  CenterOfMassUnits=in  MomentsOfInertia=smiData.Solid(19).MoI  MomentsOfInertiaUnits=kg*in^2  ProductsOfInertia=smiData.Solid(19).PoI  ProductsOfInertiaUnits=kg*in^2  GraphicType=FromGeometry  MarkerShape=Sphere  MarkerSize=10  GraphicVisPropType=SimpleVisualProperties  GraphicDiffuseColor=smiData.Solid(19).color  GraphicOpacity=smiData.Solid(19).opacity  GraphicSpecularColor=[0.5 0.5 0.5 1.0]  GraphicAmbientColor=[0.15 0.15 0.15 1.0]  GraphicEmissiveColor=[0.0 0.0 0.0 1.0]  GraphicShininess=75  DoExposeReferenceFrame=on  SerializedFrames=<Frames/>
  Transform2 : sm_lib/Frames and Transforms/Rigid Transform  RotationMethod=ArbitraryAxis  FollAlignAxisA=+X  BaseAlignAxisA=+Y  FollAlignAxisB=+Y  BaseAlignAxisB=+Z  RotationStandardAxis=+Z  RotationAngle=smiData.RigidTransform(229).angle  RotationAngleUnits=rad  RotationArbitraryAxis=smiData.RigidTransform(229).axis  RotationSequenceAxes=FollowerAxes  RotationSequence=XYX  RotationSequenceAngles=[0 0 0]  RotationSequenceAnglesUnits=deg  RotationMatrix=[1 0 0;0 1 0;0 0 1]  Quaternion=[1 0 0 0]  TranslationMethod=Cartesian  TranslationCartesianOffset=smiData.RigidTransform(229).translation  TranslationCartesianOffsetUnits=mm  TranslationStandardAxis=+Z  TranslationStandardOffset=0  TranslationStandardOffsetUnits=m  TranslationROffset=0  TranslationROffsetUnits=m  TranslationThetaOffset=0  TranslationThetaOffsetUnits=deg  TranslationZOffset=0  TranslationZOffsetUnits=m
  Transform3 : sm_lib/Frames and Transforms/Rigid Transform  RotationMethod=ArbitraryAxis  FollAlignAxisA=+X  BaseAlignAxisA=+Y  FollAlignAxisB=+Y  BaseAlignAxisB=+Z  RotationStandardAxis=+Z  RotationAngle=smiData.RigidTransform(230).angle  RotationAngleUnits=rad  RotationArbitraryAxis=smiData.RigidTransform(230).axis  RotationSequenceAxes=FollowerAxes  RotationSequence=XYX  RotationSequenceAngles=[0 0 0]  RotationSequenceAnglesUnits=deg  RotationMatrix=[1 0 0;0 1 0;0 0 1]  Quaternion=[1 0 0 0]  TranslationMethod=Cartesian  TranslationCartesianOffset=smiData.RigidTransform(230).translation  TranslationCartesianOffsetUnits=mm  TranslationStandardAxis=+Z  TranslationStandardOffset=0  TranslationStandardOffsetUnits=m  TranslationROffset=0  TranslationROffsetUnits=m  TranslationThetaOffset=0  TranslationThetaOffsetUnits=deg  TranslationZOffset=0  TranslationZOffsetUnits=m
  Transform4 : sm_lib/Frames and Transforms/Rigid Transform  RotationMethod=ArbitraryAxis  FollAlignAxisA=+X  BaseAlignAxisA=+Y  FollAlignAxisB=+Y  BaseAlignAxisB=+Z  RotationStandardAxis=+Z  RotationAngle=smiData.RigidTransform(231).angle  RotationAngleUnits=rad  RotationArbitraryAxis=smiData.RigidTransform(231).axis  RotationSequenceAxes=FollowerAxes  RotationSequence=XYX  RotationSequenceAngles=[0 0 0]  RotationSequenceAnglesUnits=deg  RotationMatrix=[1 0 0;0 1 0;0 0 1]  Quaternion=[1 0 0 0]  TranslationMethod=Cartesian  TranslationCartesianOffset=smiData.RigidTransform(231).translation  TranslationCartesianOffsetUnits=mm  TranslationStandardAxis=+Z  TranslationStandardOffset=0  TranslationStandardOffsetUnits=m  TranslationROffset=0  TranslationROffsetUnits=m  TranslationThetaOffset=0  TranslationThetaOffsetUnits=deg  TranslationZOffset=0  TranslationZOffsetUnits=m
  B : PMIOPort  Side=Left
  T : PMIOPort  Port=2  Side=Right
  connections:
  Transform3/LConn1 -- Transform4/LConn1 -- ReferenceFrame/RConn1 -- Transform2/LConn1
  Solid2/RConn1 -- Transform2/RConn1
  Solid/RConn1 -- Transform3/RConn1
  Solid1/RConn1 -- Transform4/RConn1
  Solid/LConn1 -- B/RConn1
  Solid1/LConn1 -- T/RConn1

== system Hexapod_PD/Spherical Joints/HeimJoint_No_Ball_1_RIGID2 ==
  ReferenceFrame : sm_lib/Frames and Transforms/Reference Frame
  Transform2 : sm_lib/Frames and Transforms/Rigid Transform  RotationMethod=ArbitraryAxis  FollAlignAxisA=+X  BaseAlignAxisA=+Y  FollAlignAxisB=+Y  BaseAlignAxisB=+Z  RotationStandardAxis=+Z  RotationAngle=smiData.RigidTransform(229).angle  RotationAngleUnits=rad  RotationArbitraryAxis=smiData.RigidTransform(229).axis  RotationSequenceAxes=FollowerAxes  RotationSequence=XYX  RotationSequenceAngles=[0 0 0]  RotationSequenceAnglesUnits=deg  RotationMatrix=[1 0 0;0 1 0;0 0 1]  Quaternion=[1 0 0 0]  TranslationMethod=Cartesian  TranslationCartesianOffset=smiData.RigidTransform(229).translation  TranslationCartesianOffsetUnits=mm  TranslationStandardAxis=+Z  TranslationStandardOffset=0  TranslationStandardOffsetUnits=m  TranslationROffset=0  TranslationROffsetUnits=m  TranslationThetaOffset=0  TranslationThetaOffsetUnits=deg  TranslationZOffset=0  TranslationZOffsetUnits=m
  Transform3 : sm_lib/Frames and Transforms/Rigid Transform  RotationMethod=ArbitraryAxis  FollAlignAxisA=+X  BaseAlignAxisA=+Y  FollAlignAxisB=+Y  BaseAlignAxisB=+Z  RotationStandardAxis=+Z  RotationAngle=smiData.RigidTransform(230).angle  RotationAngleUnits=rad  RotationArbitraryAxis=smiData.RigidTransform(230).axis  RotationSequenceAxes=FollowerAxes  RotationSequence=XYX  RotationSequenceAngles=[0 0 0]  RotationSequenceAnglesUnits=deg  RotationMatrix=[1 0 0;0 1 0;0 0 1]  Quaternion=[1 0 0 0]  TranslationMethod=Cartesian  TranslationCartesianOffset=smiData.RigidTransform(230).translation  TranslationCartesianOffsetUnits=mm  TranslationStandardAxis=+Z  TranslationStandardOffset=0  TranslationStandardOffsetUnits=m  TranslationROffset=0  TranslationROffsetUnits=m  TranslationThetaOffset=0  TranslationThetaOffsetUnits=deg  TranslationZOffset=0  TranslationZOffsetUnits=m
  Transform4 : sm_lib/Frames and Transforms/Rigid Transform  RotationMethod=ArbitraryAxis  FollAlignAxisA=+X  BaseAlignAxisA=+Y  FollAlignAxisB=+Y  BaseAlignAxisB=+Z  RotationStandardAxis=+Z  RotationAngle=smiData.RigidTransform(231).angle  RotationAngleUnits=rad  RotationArbitraryAxis=smiData.RigidTransform(231).axis  RotationSequenceAxes=FollowerAxes  RotationSequence=XYX  RotationSequenceAngles=[0 0 0]  RotationSequenceAnglesUnits=deg  RotationMatrix=[1 0 0;0 1 0;0 0 1]  Quaternion=[1 0 0 0]  TranslationMethod=Cartesian  TranslationCartesianOffset=smiData.RigidTransform(231).translation  TranslationCartesianOffsetUnits=mm  TranslationStandardAxis=+Z  TranslationStandardOffset=0  TranslationStandardOffsetUnits=m  TranslationROffset=0  TranslationROffsetUnits=m  TranslationThetaOffset=0  TranslationThetaOffsetUnits=deg  TranslationZOffset=0  TranslationZOffsetUnits=m
  x6960T431_Super_Swivel_Ball_Joint_Rod_End_No_Ball_1_RIGID : Subsystem
  x6960T432_Super_Swivel_Ball_Joint_Rod_End_No_Ball_1_RIGID : Subsystem
  x8422N111_18_8_Stainless_Steel_Turnbuckle_Style_Connecting_Rod_1_RIGID : Subsystem
  B : PMIOPort  Side=Left
  T : PMIOPort  Port=2  Side=Right
  connections:
  Transform3/LConn1 -- Transform4/LConn1 -- ReferenceFrame/RConn1 -- Transform2/LConn1
  Transform2/RConn1 -- x8422N111_18_8_Stainless_Steel_Turnbuckle_Style_Connecting_Rod_1_RIGID/LConn1
  Transform3/RConn1 -- x6960T431_Super_Swivel_Ball_Joint_Rod_End_No_Ball_1_RIGID/LConn1
  Transform4/RConn1 -- x6960T432_Super_Swivel_Ball_Joint_Rod_End_No_Ball_1_RIGID/LConn1
  B/RConn1 -- x6960T431_Super_Swivel_Ball_Joint_Rod_End_No_Ball_1_RIGID/LConn2
  T/RConn1 -- x6960T432_Super_Swivel_Ball_Joint_Rod_End_No_Ball_1_RIGID/LConn2

== system Hexapod_PD/Spherical Joints/HeimJoint_No_Ball_1_RIGID3 ==
  ReferenceFrame : sm_lib/Frames and Transforms/Reference Frame
  Transform2 : sm_lib/Frames and Transforms/Rigid Transform  RotationMethod=ArbitraryAxis  FollAlignAxisA=+X  BaseAlignAxisA=+Y  FollAlignAxisB=+Y  BaseAlignAxisB=+Z  RotationStandardAxis=+Z  RotationAngle=smiData.RigidTransform(229).angle  RotationAngleUnits=rad  RotationArbitraryAxis=smiData.RigidTransform(229).axis  RotationSequenceAxes=FollowerAxes  RotationSequence=XYX  RotationSequenceAngles=[0 0 0]  RotationSequenceAnglesUnits=deg  RotationMatrix=[1 0 0;0 1 0;0 0 1]  Quaternion=[1 0 0 0]  TranslationMethod=Cartesian  TranslationCartesianOffset=smiData.RigidTransform(229).translation  TranslationCartesianOffsetUnits=mm  TranslationStandardAxis=+Z  TranslationStandardOffset=0  TranslationStandardOffsetUnits=m  TranslationROffset=0  TranslationROffsetUnits=m  TranslationThetaOffset=0  TranslationThetaOffsetUnits=deg  TranslationZOffset=0  TranslationZOffsetUnits=m
  Transform3 : sm_lib/Frames and Transforms/Rigid Transform  RotationMethod=ArbitraryAxis  FollAlignAxisA=+X  BaseAlignAxisA=+Y  FollAlignAxisB=+Y  BaseAlignAxisB=+Z  RotationStandardAxis=+Z  RotationAngle=smiData.RigidTransform(230).angle  RotationAngleUnits=rad  RotationArbitraryAxis=smiData.RigidTransform(230).axis  RotationSequenceAxes=FollowerAxes  RotationSequence=XYX  RotationSequenceAngles=[0 0 0]  RotationSequenceAnglesUnits=deg  RotationMatrix=[1 0 0;0 1 0;0 0 1]  Quaternion=[1 0 0 0]  TranslationMethod=Cartesian  TranslationCartesianOffset=smiData.RigidTransform(230).translation  TranslationCartesianOffsetUnits=mm  TranslationStandardAxis=+Z  TranslationStandardOffset=0  TranslationStandardOffsetUnits=m  TranslationROffset=0  TranslationROffsetUnits=m  TranslationThetaOffset=0  TranslationThetaOffsetUnits=deg  TranslationZOffset=0  TranslationZOffsetUnits=m
  Transform4 : sm_lib/Frames and Transforms/Rigid Transform  RotationMethod=ArbitraryAxis  FollAlignAxisA=+X  BaseAlignAxisA=+Y  FollAlignAxisB=+Y  BaseAlignAxisB=+Z  RotationStandardAxis=+Z  RotationAngle=smiData.RigidTransform(231).angle  RotationAngleUnits=rad  RotationArbitraryAxis=smiData.RigidTransform(231).axis  RotationSequenceAxes=FollowerAxes  RotationSequence=XYX  RotationSequenceAngles=[0 0 0]  RotationSequenceAnglesUnits=deg  RotationMatrix=[1 0 0;0 1 0;0 0 1]  Quaternion=[1 0 0 0]  TranslationMethod=Cartesian  TranslationCartesianOffset=smiData.RigidTransform(231).translation  TranslationCartesianOffsetUnits=mm  TranslationStandardAxis=+Z  TranslationStandardOffset=0  TranslationStandardOffsetUnits=m  TranslationROffset=0  TranslationROffsetUnits=m  TranslationThetaOffset=0  TranslationThetaOffsetUnits=deg  TranslationZOffset=0  TranslationZOffsetUnits=m
  x6960T431_Super_Swivel_Ball_Joint_Rod_End_No_Ball_1_RIGID : Subsystem
  x6960T432_Super_Swivel_Ball_Joint_Rod_End_No_Ball_1_RIGID : Subsystem
  x8422N111_18_8_Stainless_Steel_Turnbuckle_Style_Connecting_Rod_1_RIGID : Subsystem
  B : PMIOPort  Side=Left
  T : PMIOPort  Port=2  Side=Right
  connections:
  Transform3/LConn1 -- Transform4/LConn1 -- ReferenceFrame/RConn1 -- Transform2/LConn1
  Transform2/RConn1 -- x8422N111_18_8_Stainless_Steel_Turnbuckle_Style_Connecting_Rod_1_RIGID/LConn1
  Transform3/RConn1 -- x6960T431_Super_Swivel_Ball_Joint_Rod_End_No_Ball_1_RIGID/LConn1
  Transform4/RConn1 -- x6960T432_Super_Swivel_Ball_Joint_Rod_End_No_Ball_1_RIGID/LConn1
  B/RConn1 -- x6960T431_Super_Swivel_Ball_Joint_Rod_End_No_Ball_1_RIGID/RConn1
  T/RConn1 -- x6960T432_Super_Swivel_Ball_Joint_Rod_End_No_Ball_1_RIGID/RConn1

== system Hexapod_PD/Spherical Joints/HeimJoint_No_Ball_1_RIGID4 ==
  ReferenceFrame : sm_lib/Frames and Transforms/Reference Frame
  Transform2 : sm_lib/Frames and Transforms/Rigid Transform  RotationMethod=ArbitraryAxis  FollAlignAxisA=+X  BaseAlignAxisA=+Y  FollAlignAxisB=+Y  BaseAlignAxisB=+Z  RotationStandardAxis=+Z  RotationAngle=smiData.RigidTransform(229).angle  RotationAngleUnits=rad  RotationArbitraryAxis=smiData.RigidTransform(229).axis  RotationSequenceAxes=FollowerAxes  RotationSequence=XYX  RotationSequenceAngles=[0 0 0]  RotationSequenceAnglesUnits=deg  RotationMatrix=[1 0 0;0 1 0;0 0 1]  Quaternion=[1 0 0 0]  TranslationMethod=Cartesian  TranslationCartesianOffset=smiData.RigidTransform(229).translation  TranslationCartesianOffsetUnits=mm  TranslationStandardAxis=+Z  TranslationStandardOffset=0  TranslationStandardOffsetUnits=m  TranslationROffset=0  TranslationROffsetUnits=m  TranslationThetaOffset=0  TranslationThetaOffsetUnits=deg  TranslationZOffset=0  TranslationZOffsetUnits=m
  Transform3 : sm_lib/Frames and Transforms/Rigid Transform  RotationMethod=ArbitraryAxis  FollAlignAxisA=+X  BaseAlignAxisA=+Y  FollAlignAxisB=+Y  BaseAlignAxisB=+Z  RotationStandardAxis=+Z  RotationAngle=smiData.RigidTransform(230).angle  RotationAngleUnits=rad  RotationArbitraryAxis=smiData.RigidTransform(230).axis  RotationSequenceAxes=FollowerAxes  RotationSequence=XYX  RotationSequenceAngles=[0 0 0]  RotationSequenceAnglesUnits=deg  RotationMatrix=[1 0 0;0 1 0;0 0 1]  Quaternion=[1 0 0 0]  TranslationMethod=Cartesian  TranslationCartesianOffset=smiData.RigidTransform(230).translation  TranslationCartesianOffsetUnits=mm  TranslationStandardAxis=+Z  TranslationStandardOffset=0  TranslationStandardOffsetUnits=m  TranslationROffset=0  TranslationROffsetUnits=m  TranslationThetaOffset=0  TranslationThetaOffsetUnits=deg  TranslationZOffset=0  TranslationZOffsetUnits=m
  Transform4 : sm_lib/Frames and Transforms/Rigid Transform  RotationMethod=ArbitraryAxis  FollAlignAxisA=+X  BaseAlignAxisA=+Y  FollAlignAxisB=+Y  BaseAlignAxisB=+Z  RotationStandardAxis=+Z  RotationAngle=smiData.RigidTransform(231).angle  RotationAngleUnits=rad  RotationArbitraryAxis=smiData.RigidTransform(231).axis  RotationSequenceAxes=FollowerAxes  RotationSequence=XYX  RotationSequenceAngles=[0 0 0]  RotationSequenceAnglesUnits=deg  RotationMatrix=[1 0 0;0 1 0;0 0 1]  Quaternion=[1 0 0 0]  TranslationMethod=Cartesian  TranslationCartesianOffset=smiData.RigidTransform(231).translation  TranslationCartesianOffsetUnits=mm  TranslationStandardAxis=+Z  TranslationStandardOffset=0  TranslationStandardOffsetUnits=m  TranslationROffset=0  TranslationROffsetUnits=m  TranslationThetaOffset=0  TranslationThetaOffsetUnits=deg  TranslationZOffset=0  TranslationZOffsetUnits=m
  x6960T431_Super_Swivel_Ball_Joint_Rod_End_No_Ball_1_RIGID : Subsystem
  x6960T432_Super_Swivel_Ball_Joint_Rod_End_No_Ball_1_RIGID : Subsystem
  x8422N111_18_8_Stainless_Steel_Turnbuckle_Style_Connecting_Rod_1_RIGID : Subsystem
  B : PMIOPort  Side=Left
  T : PMIOPort  Port=2  Side=Right
  connections:
  Transform3/LConn1 -- Transform4/LConn1 -- ReferenceFrame/RConn1 -- Transform2/LConn1
  Transform2/RConn1 -- x8422N111_18_8_Stainless_Steel_Turnbuckle_Style_Connecting_Rod_1_RIGID/LConn1
  Transform3/RConn1 -- x6960T431_Super_Swivel_Ball_Joint_Rod_End_No_Ball_1_RIGID/LConn1
  Transform4/RConn1 -- x6960T432_Super_Swivel_Ball_Joint_Rod_End_No_Ball_1_RIGID/LConn1
  B/RConn1 -- x6960T431_Super_Swivel_Ball_Joint_Rod_End_No_Ball_1_RIGID/LConn2
  T/RConn1 -- x6960T432_Super_Swivel_Ball_Joint_Rod_End_No_Ball_1_RIGID/LConn2
